simulink model "DualBuckPPS22016_define"  (R2024b)
settings: Solver=ode45  StartTime=0.0  StopTime=0.5  RelTol=1e-3
model workspace (MAT data in the model file):
  D = 50
  T = 0.0333333333333
undefined symbols (not defined in the file): C, D_T_DOWN_Given, D_T_UP_Given, DiscIntNeverNeededParam, P, R, T_pulse, TP
libraries: spsOnDelayLib x27, dspsnks4 x12, dspfdesign x11, spsCurrentMeasurementLib x11, spsSeriesRLCBranchLib x8, spsMosfetLib x4, slpidlib x4, spsVoltageMeasurementLib x4, simulink x3, spsControlledCurrentSourceLib x1, spsDCVoltageSourceLib x1, spspowerguiLib x1
(part 1 of 2)
settings Model: SimulationMode=accelerator  Creator=10474  LastModifiedBy=admin
settings SolverCC: AlgebraicLoopSolver=TrustRegion
settings OptimizationCC: ReuseModelBlockBuffer=off
settings DebuggingCC: UnconnectedInputMsg=warning  UnconnectedOutputMsg=warning  UnconnectedLineMsg=warning  ArithmeticOperatorsInVariantConditions=warning
settings ModelReferenceCC: EnableRefExpFcnMdlSchedulingChecks=on
settings SFSimCC: CustomCodeUndefinedFunction=UseInterfaceOnly
settings RTWCC: GPUComputeCapability=3.5
settings CodeAppCC: StateflowObjectComments=on

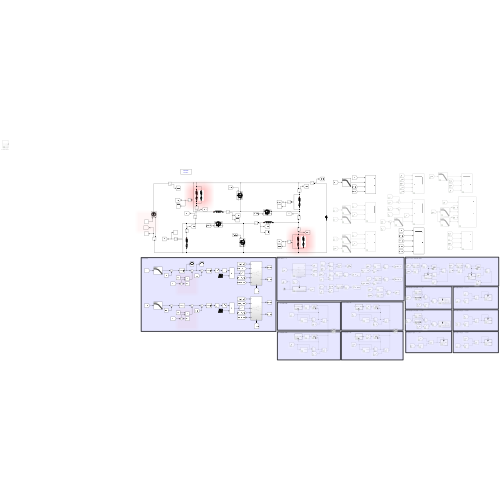
[thumbnail: Simulink's stored preview of the top-level diagram]
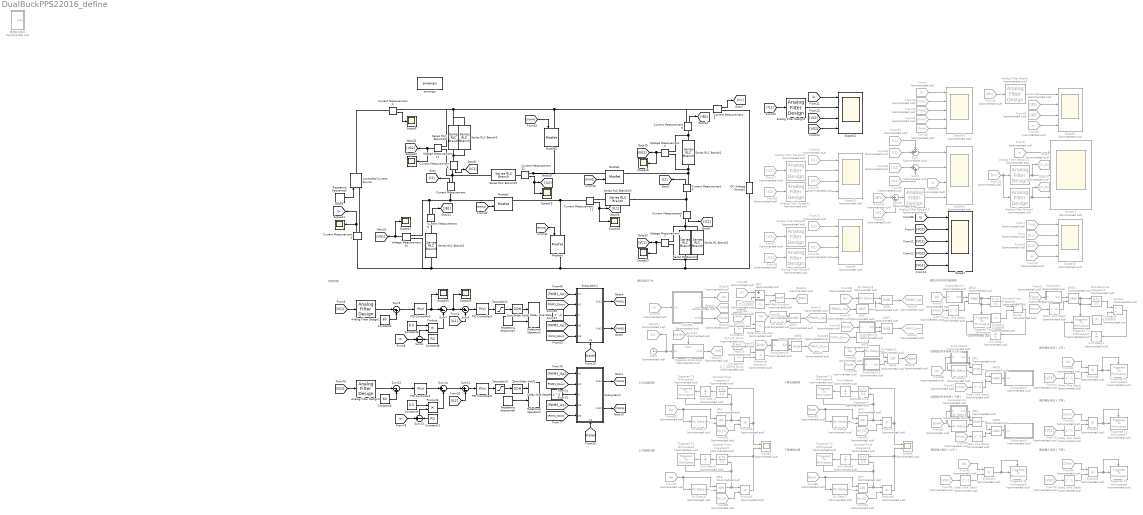
== system DualBuckPPS22016_define ==
  note: 控制回路
  note: 上升尖峰获取
  note: 上升滤除尖峰
  note: 下降尖峰获取
  note: 下降滤除尖峰
  note: 切回稳态开关采样（上升）
  note: 瞬态开关序列均值获取
  note: 切回稳态开关采样（下降）
  note: 瞬态波形产生
  note: 瞬态输入电压（下降）
  note: 瞬态输出电压（下降）
  note: 瞬态输出电压（上升）
  note: 瞬态输入电压（上升）
  AND{1..8} (8 alike) : Logic  Commented=on  IconShape=distinctive  AllPortsSameDT=off  OutDataTypeStr=boolean
  AND9 : Logic  Commented=on  Operator=OR  IconShape=distinctive  AllPortsSameDT=off  OutDataTypeStr=boolean
  Add : Sum  Commented=on  Inputs=+-
  Analog Filter Design{,5..6,10..12} (6 alike) : dspfdesign/Analog Filter Design  Commented=on  method=Butterworth  filttype=Lowpass  N=8  Wlo=2*pi*5000  Whi=80  Rp=2  Rs=40
  Analog Filter Design1 : dspfdesign/Analog Filter Design  Commented=on  method=Butterworth  filttype=Lowpass  N=2  Wlo=2*pi*1000  Whi=80  Rp=2  Rs=40
  Analog Filter Design13 : dspfdesign/Analog Filter Design  Commented=on  method=Butterworth  filttype=Lowpass  N=2  Wlo=2*pi*10000  Whi=80  Rp=2  Rs=40
  Analog Filter Design2 : dspfdesign/Analog Filter Design  method=Butterworth  filttype=Lowpass  N=1  Wlo=10  Whi=80  Rp=2  Rs=40
  Analog Filter Design3 : dspfdesign/Analog Filter Design  method=Butterworth  filttype=Lowpass  N=1  Wlo=10  Whi=80  Rp=2  Rs=40
  Analog Filter Design9 : dspfdesign/Analog Filter Design  method=Butterworth  filttype=Lowpass  N=8  Wlo=2*pi*5000  Whi=80  Rp=2  Rs=40
  Clock : Clock  Commented=on
  Constant : Constant  Commented=on  Value=1/100000
  Constant1 : Constant  Commented=on  Value=1/100000
  Constant10 : Constant  Commented=on  Value=D_T_DOWN_Given
  Constant11 : Constant  Value=P/2
  Constant2 : Constant  Commented=on  Value=D_T_UP_Given
  Constant3 : Constant  Value=60
  Constant4 : Constant  Value=60
  Constant5 : Constant  Commented=on  Value=1/100000
  Constant6 : Constant  Value=0.5
  Constant8 : Constant  Value=P/2
  Constant9 : Constant  Value=0.5
  Controlled Current Source : spsControlledCurrentSourceLib/Controlled Current Source  Initialize=on  Source_Type=DC  Amplitude=0  Phase=0  Frequency=0  Measurements=None
  Current Measurement{,1..8,11..12} (11 alike) : spsCurrentMeasurementLib/Current Measurement  PhasorSimulation=off  OutputType=Complex  PSBequivalent=0
  DC Voltage Source1 : spsDCVoltageSourceLib/DC Voltage Source  Amplitude=270  Measurements=None
  Delay One Step : Delay  DelayLength=1
  Delay One Step1 : Delay  Commented=on
  Delay One Step{2..3,5..8} (6 alike) : Delay  Commented=on  DelayLength=1
  Delay One Step4 : Delay  Commented=on
  Delay One Step9 : Delay  DelayLength=1
  Discrete-Time Integrator{,1,3..6} (6 alike) : DiscreteIntegrator  Commented=on  ExternalReset=falling  SampleTime=-1  ICPrevOutput=DiscIntNeverNeededParam  ICPrevScaledInput=DiscIntNeverNeededParam
  Divide : Product  Commented=on  Inputs=*/
  Divide1 : Product  Commented=on  Inputs=*/
  From : From  Commented=on  GotoTag=IL1
  From10 : From  Commented=on  GotoTag=IL2
  From{2,9,14,37,39,47} (6 alike) : From  Commented=on  GotoTag=io  TagVisibility=global
  From{15,25,29,41} (4 alike) : From  Commented=on  GotoTag=I1
  From16 : From  Commented=on  GotoTag=I2
  From17 : From  Commented=on  GotoTag=IC1
  From18 : From  Commented=on  GotoTag=IC2
  From19 : From  Commented=on  GotoTag=Iin
  From26 : From  Commented=on  GotoTag=I2
  From27 : From  Commented=on  GotoTag=IL1
  From28 : From  Commented=on  GotoTag=IL2
  From{3,42,55,61,66} (5 alike) : From  Commented=on  GotoTag=PWM1
  From34 : From  Commented=on  GotoTag=I2
  From35 : From  Commented=on  GotoTag=IL2
  From36 : From  Commented=on  GotoTag=IL1
  From38 : From  Commented=on  GotoTag=IB2
  From40 : From  Commented=on  GotoTag=IB1
  From43 : From  Commented=on  GotoTag=PWM2
  From44 : From  Commented=on  GotoTag=PWM3
  From45 : From  Commented=on  GotoTag=PWM4
  From46 : From  Commented=on  GotoTag=IB1
  From48 : From  Commented=on  GotoTag=IB1
  From{5,58,60,72,83,88,90,94,96} (9 alike) : From  Commented=on  GotoTag=Down  TagVisibility=global
  From54 : From  Commented=on  GotoTag=VC1
  From{56,67..69,81..82,87,92,95} (9 alike) : From  Commented=on  GotoTag=Up  TagVisibility=global
  From57 : From  Commented=on  GotoTag=PWM1_Up
  From59 : From  Commented=on  GotoTag=PWM1_Down  TagVisibility=global
  From63 : From  Commented=on  GotoTag=t0
  From64 : From  Commented=on  GotoTag=State1  TagVisibility=global
  From65 : From  Commented=on  GotoTag=t
  From7 : From  Commented=on  GotoTag=Iin
  From71 : From  Commented=on  GotoTag=MW
  From73 : From  Commented=on  GotoTag=MW
  From79 : From  Commented=on  GotoTag=VC1
  From80 : From  Commented=on  GotoTag=Iin_f1
  From84 : From  Commented=on  GotoTag=Iin_f2
  From85 : From  Commented=on  GotoTag=Iin_f1
  From89 : From  Commented=on  GotoTag=Iin_f2
  From91 : From  Commented=on  GotoTag=VG1
  From93 : From  Commented=on  GotoTag=VG1
  Goto10 : Goto  Commented=on  GotoTag=Up  TagVisibility=global
  Goto11 : Goto  Commented=on  GotoTag=State  TagVisibility=global
  Goto13 : Goto  Commented=on  GotoTag=Down  TagVisibility=global
  Goto15 : Goto  Commented=on  GotoTag=Iin_f2
  Goto16 : Goto  Commented=on  GotoTag=PWM2_Up
  Goto17 : Goto  Commented=on  GotoTag=PWM2_Down
  Goto18 : Goto  Commented=on  GotoTag=State1  TagVisibility=global
  Goto20 : Goto  Commented=on  GotoTag=t0
  Goto21 : Goto  Commented=on  GotoTag=t
  Goto22 : Goto  Commented=on  GotoTag=PWM1_Down  TagVisibility=global
  Goto23 : Goto  Commented=on  GotoTag=PWM1_Up
  Goto24 : Goto  Commented=on  GotoTag=MW
  Goto3 : Goto  Commented=on  GotoTag=Iin_f1
  Math Function : Math  Commented=on  Operator=mod
  Mosfet{1..4} (4 alike) : spsMosfetLib/Mosfet  Ron=53e-3  Lon=0  Rd=0.001  Vfd=2  IC=0  Rs=1e5  Cs=inf  Measurements=on
  NOT7 : Logic  Commented=on  Operator=NOT  IconShape=distinctive  AllPortsSameDT=off  OutDataTypeStr=boolean
  NOT8 : Logic  Commented=on  Operator=NOT  IconShape=distinctive  AllPortsSameDT=off  OutDataTypeStr=boolean
  OR2 : Logic  Commented=on  Operator=XOR  IconShape=distinctive  AllPortsSameDT=off  OutDataTypeStr=boolean
  OR3 : Logic  Commented=on  Operator=XOR  IconShape=distinctive  AllPortsSameDT=off  OutDataTypeStr=boolean
  OR{4..7} (4 alike) : Logic  Commented=on  Operator=OR  IconShape=distinctive  AllPortsSameDT=off  OutDataTypeStr=boolean
  On Delay1 : spsOnDelayLib/On Delay  Commented=on  DelayType=Off delay  delay=ceil(TP*1e5)*1e-5-TP  ic=0  Ts=0
  On Delay11 : spsOnDelayLib/On Delay  Commented=on  DelayType=Off delay  delay=ceil(TP*1e5)*1e-5-TP  ic=0  Ts=0
  On Delay12 : spsOnDelayLib/On Delay  Commented=on  DelayType=Off delay  delay=ceil(TP*1e5)*1e-5-TP  ic=0  Ts=0
  On Delay3 : spsOnDelayLib/On Delay  Commented=on  DelayType=Off delay  delay=30e-6  ic=0  Ts=0
  On Delay{4..7} (4 alike) : spsOnDelayLib/On Delay  Commented=on  DelayType=Off delay  delay=TP  ic=0  Ts=0
  On Delay9 : spsOnDelayLib/On Delay  Commented=on  DelayType=Off delay  delay=30e-6  ic=0  Ts=0
  PID Controller1 : slpidlib/PID Controller  Controller=PI  Form=Parallel  TimeDomain=Discrete-time  UseExternalTs=off  SampleTime=-1  IntegratorMethod=Forward Euler  FilterMethod=Forward Euler  ControllerParametersSource=internal  P=0.15  I=0.5  UseKiTs=off  D=0  UseExternalDerivativeSource=off  N=100  UseFilter=on  TunerSelectOption=Transfer Function Based (PID Tuner App)  InitialConditionSource=internal  InitialConditionForIntegrator=0  InitialConditionForFilter=0  DifferentiatorICPrevScaledInput=0  ExternalReset=none  TrackingMode=off  Kt=1  LimitOutput=on  SatLimitsSource=internal  UpperSaturationLimit=10  LowerSaturationLimit=-10  LinearizeAsGain=on  AntiWindupMode=none  Kb=1  LimitIntegrator=off  UpperIntegratorSaturationLimit=inf  LowerIntegratorSaturationLimit=-inf  POutMin=[]  POutMax=[]  IOutMin=[]  IOutMax=[]  DOutMin=[]  DOutMax=[]  NOutMin=[]  NOutMax=[]  SumOutMin=[]  SumOutMax=[]  SaturationOutMin=[]  SaturationOutMax=[]  PParamMin=[]  PParamMax=[]  IParamMin=[]  IParamMax=[]  DParamMin=[]  DParamMax=[]  NParamMin=[]  NParamMax=[]  KbParamMin=[]  KbParamMax=[]  KtParamMin=[]  KtParamMax=[]  KbOutMin=[]  KbOutMax=[]  KtOutMin=[]  KtOutMax=[]  IntegratorOutMin=[]  IntegratorOutMax=[]  FilterOutMin=[]  FilterOutMax=[]  SumI1OutMin=[]  SumI1OutMax=[]  SumI2OutMin=[]  SumI2OutMax=[]  SumI3OutMin=[]  SumI3OutMax=[]  SumI4OutMin=[]  SumI4OutMax=[]  SumDOutMin=[]  SumDOutMax=[]  DifferentiatorOutMin=[]  DifferentiatorOutMax=[]  FilterDiffOutCoefMin=[]  FilterDiffOutCoefMax=[]  ReciprocalOutMin=[]  ReciprocalOutMax=[]  SumDenOutMin=[]  SumDenOutMax=[]  SumNumOutMin=[]  SumNumOutMax=[]  DivideOutMin=[]  DivideOutMax=[]  UdiffTsProdOutMin=[]  UdiffTsProdOutMax=[]  NTsProdOutMin=[]  NTsProdOutMax=[]  UintegralTsProdOutMin=[]  UintegralTsProdOutMax=[]  UngainTsProdOutMin=[]  UngainTsProdOutMax=[]  ClampingZeroOutDataTypeStr=Inherit: Inherit via back propagation  ClampingZeroOutMin=[]  ClampingZeroOutMax=[]  FilterDenConstantOutDataTypeStr=Inherit: Inherit via back propagation  FilterDenConstantOutMin=[]  FilterDenConstantOutMax=[]  PCopyOutDataTypeStr=Inherit: Inherit via back propagation  PCopyOutMin=[]  PCopyOutMax=[]  NCopyOutDataTypeStr=Inherit: Inherit via back propagation  NCopyOutMin=[]  NCopyOutMax=[]  IntegratorContinuousStateAttributes=''  IntegratorStateMustResolveToSignalObject=off  IntegratorRTWStateStorageClass=Auto  FilterContinuousStateAttributes=''  FilterStateMustResolveToSignalObject=off  FilterRTWStateStorageClass=Auto  ParallelPVariant=InternalParameters  IdealPVariant=Disabled  IVariant=InternalParameters  DVariant=Disabled  IntegratorVariant=Discrete  SatVariant=Enabled  AWVariant=Passthrough  PCopyVariant=Disabled  TRVariant=Disabled  FdbkBlocksVariant=Forward  IdealPFdbkVariant=Disabled  SatFdbkVariant=Disabled  DerivativeFilterVariant=Disabled  NVariant=Disabled  NCopyVariant=Disabled_SignalSpec  FilterICVariant=Disabled  IntegratorICVariant=InternalICs  ExternalResetVariant=Disabled  TRSumVariant=Passthrough  SumFdbkVariant=Disabled  SumVariant=Sum_PI  TsampFilterVariant=InternalTs  TsampNgainVariant=Passthrough  TsampIntegralVariant=Disabled_SignalSpec  ExternalSaturationOutDataTypeStr=Inherit: Same as second input  DerivativeSourceVariant=Disabled  PreIntVariant=InternalPreInt
  PID Controller3 : slpidlib/PID Controller  Controller=PI  Form=Parallel  TimeDomain=Discrete-time  UseExternalTs=off  SampleTime=-1  IntegratorMethod=Forward Euler  FilterMethod=Forward Euler  ControllerParametersSource=internal  P=0.2  I=2  UseKiTs=off  D=0  UseExternalDerivativeSource=off  N=100  UseFilter=on  TunerSelectOption=Transfer Function Based (PID Tuner App)  InitialConditionSource=internal  InitialConditionForIntegrator=0  InitialConditionForFilter=0  DifferentiatorICPrevScaledInput=0  ExternalReset=none  TrackingMode=off  Kt=1  LimitOutput=on  SatLimitsSource=internal  UpperSaturationLimit=0.98  LowerSaturationLimit=0  LinearizeAsGain=on  AntiWindupMode=none  Kb=1  LimitIntegrator=off  UpperIntegratorSaturationLimit=inf  LowerIntegratorSaturationLimit=-inf  POutMin=[]  POutMax=[]  IOutMin=[]  IOutMax=[]  DOutMin=[]  DOutMax=[]  NOutMin=[]  NOutMax=[]  SumOutMin=[]  SumOutMax=[]  SaturationOutMin=[]  SaturationOutMax=[]  PParamMin=[]  PParamMax=[]  IParamMin=[]  IParamMax=[]  DParamMin=[]  DParamMax=[]  NParamMin=[]  NParamMax=[]  KbParamMin=[]  KbParamMax=[]  KtParamMin=[]  KtParamMax=[]  KbOutMin=[]  KbOutMax=[]  KtOutMin=[]  KtOutMax=[]  IntegratorOutMin=[]  IntegratorOutMax=[]  FilterOutMin=[]  FilterOutMax=[]  SumI1OutMin=[]  SumI1OutMax=[]  SumI2OutMin=[]  SumI2OutMax=[]  SumI3OutMin=[]  SumI3OutMax=[]  SumI4OutMin=[]  SumI4OutMax=[]  SumDOutMin=[]  SumDOutMax=[]  DifferentiatorOutMin=[]  DifferentiatorOutMax=[]  FilterDiffOutCoefMin=[]  FilterDiffOutCoefMax=[]  ReciprocalOutMin=[]  ReciprocalOutMax=[]  SumDenOutMin=[]  SumDenOutMax=[]  SumNumOutMin=[]  SumNumOutMax=[]  DivideOutMin=[]  DivideOutMax=[]  UdiffTsProdOutMin=[]  UdiffTsProdOutMax=[]  NTsProdOutMin=[]  NTsProdOutMax=[]  UintegralTsProdOutMin=[]  UintegralTsProdOutMax=[]  UngainTsProdOutMin=[]  UngainTsProdOutMax=[]  ClampingZeroOutDataTypeStr=Inherit: Inherit via back propagation  ClampingZeroOutMin=[]  ClampingZeroOutMax=[]  FilterDenConstantOutDataTypeStr=Inherit: Inherit via back propagation  FilterDenConstantOutMin=[]  FilterDenConstantOutMax=[]  PCopyOutDataTypeStr=Inherit: Inherit via back propagation  PCopyOutMin=[]  PCopyOutMax=[]  NCopyOutDataTypeStr=Inherit: Inherit via back propagation  NCopyOutMin=[]  NCopyOutMax=[]  IntegratorContinuousStateAttributes=''  IntegratorStateMustResolveToSignalObject=off  IntegratorRTWStateStorageClass=Auto  FilterContinuousStateAttributes=''  FilterStateMustResolveToSignalObject=off  FilterRTWStateStorageClass=Auto  ParallelPVariant=InternalParameters  IdealPVariant=Disabled  IVariant=InternalParameters  DVariant=Disabled  IntegratorVariant=Discrete  SatVariant=Enabled  AWVariant=Passthrough  PCopyVariant=Disabled  TRVariant=Disabled  FdbkBlocksVariant=Forward  IdealPFdbkVariant=Disabled  SatFdbkVariant=Disabled  DerivativeFilterVariant=Disabled  NVariant=Disabled  NCopyVariant=Disabled_SignalSpec  FilterICVariant=Disabled  IntegratorICVariant=InternalICs  ExternalResetVariant=Disabled  TRSumVariant=Passthrough  SumFdbkVariant=Disabled  SumVariant=Sum_PI  TsampFilterVariant=InternalTs  TsampNgainVariant=Passthrough  TsampIntegralVariant=Disabled_SignalSpec  ExternalSaturationOutDataTypeStr=Inherit: Same as second input  DerivativeSourceVariant=Disabled  PreIntVariant=InternalPreInt
  PID Controller4 : slpidlib/PID Controller  Controller=PI  Form=Parallel  TimeDomain=Discrete-time  UseExternalTs=off  SampleTime=-1  IntegratorMethod=Forward Euler  FilterMethod=Forward Euler  ControllerParametersSource=internal  P=0.15  I=0.5  UseKiTs=off  D=0  UseExternalDerivativeSource=off  N=100  UseFilter=on  TunerSelectOption=Transfer Function Based (PID Tuner App)  InitialConditionSource=internal  InitialConditionForIntegrator=0  InitialConditionForFilter=0  DifferentiatorICPrevScaledInput=0  ExternalReset=none  TrackingMode=off  Kt=1  LimitOutput=off  SatLimitsSource=internal  UpperSaturationLimit=1  LowerSaturationLimit=-1  LinearizeAsGain=on  AntiWindupMode=none  Kb=1  LimitIntegrator=off  UpperIntegratorSaturationLimit=inf  LowerIntegratorSaturationLimit=-inf  POutMin=[]  POutMax=[]  IOutMin=[]  IOutMax=[]  DOutMin=[]  DOutMax=[]  NOutMin=[]  NOutMax=[]  SumOutMin=[]  SumOutMax=[]  SaturationOutMin=[]  SaturationOutMax=[]  PParamMin=[]  PParamMax=[]  IParamMin=[]  IParamMax=[]  DParamMin=[]  DParamMax=[]  NParamMin=[]  NParamMax=[]  KbParamMin=[]  KbParamMax=[]  KtParamMin=[]  KtParamMax=[]  KbOutMin=[]  KbOutMax=[]  KtOutMin=[]  KtOutMax=[]  IntegratorOutMin=[]  IntegratorOutMax=[]  FilterOutMin=[]  FilterOutMax=[]  SumI1OutMin=[]  SumI1OutMax=[]  SumI2OutMin=[]  SumI2OutMax=[]  SumI3OutMin=[]  SumI3OutMax=[]  SumI4OutMin=[]  SumI4OutMax=[]  SumDOutMin=[]  SumDOutMax=[]  DifferentiatorOutMin=[]  DifferentiatorOutMax=[]  FilterDiffOutCoefMin=[]  FilterDiffOutCoefMax=[]  ReciprocalOutMin=[]  ReciprocalOutMax=[]  SumDenOutMin=[]  SumDenOutMax=[]  SumNumOutMin=[]  SumNumOutMax=[]  DivideOutMin=[]  DivideOutMax=[]  UdiffTsProdOutMin=[]  UdiffTsProdOutMax=[]  NTsProdOutMin=[]  NTsProdOutMax=[]  UintegralTsProdOutMin=[]  UintegralTsProdOutMax=[]  UngainTsProdOutMin=[]  UngainTsProdOutMax=[]  ClampingZeroOutDataTypeStr=Inherit: Inherit via back propagation  ClampingZeroOutMin=[]  ClampingZeroOutMax=[]  FilterDenConstantOutDataTypeStr=Inherit: Inherit via back propagation  FilterDenConstantOutMin=[]  FilterDenConstantOutMax=[]  PCopyOutDataTypeStr=Inherit: Inherit via back propagation  PCopyOutMin=[]  PCopyOutMax=[]  NCopyOutDataTypeStr=Inherit: Inherit via back propagation  NCopyOutMin=[]  NCopyOutMax=[]  IntegratorContinuousStateAttributes=''  IntegratorStateMustResolveToSignalObject=off  IntegratorRTWStateStorageClass=Auto  FilterContinuousStateAttributes=''  FilterStateMustResolveToSignalObject=off  FilterRTWStateStorageClass=Auto  ParallelPVariant=InternalParameters  IdealPVariant=Disabled  IVariant=InternalParameters  DVariant=Disabled  IntegratorVariant=Discrete  SatVariant=Disabled  AWVariant=Passthrough  PCopyVariant=Disabled  TRVariant=Disabled  FdbkBlocksVariant=Forward  IdealPFdbkVariant=Disabled  SatFdbkVariant=Disabled  DerivativeFilterVariant=Disabled  NVariant=Disabled  NCopyVariant=Disabled_SignalSpec  FilterICVariant=Disabled  IntegratorICVariant=InternalICs  ExternalResetVariant=Disabled  TRSumVariant=Passthrough  SumFdbkVariant=Disabled  SumVariant=Sum_PI  TsampFilterVariant=InternalTs  TsampNgainVariant=Passthrough  TsampIntegralVariant=Disabled_SignalSpec  ExternalSaturationOutDataTypeStr=Inherit: Same as second input  DerivativeSourceVariant=Disabled  PreIntVariant=InternalPreInt
  PID Controller5 : slpidlib/PID Controller  Controller=PI  Form=Parallel  TimeDomain=Discrete-time  UseExternalTs=off  SampleTime=-1  IntegratorMethod=Forward Euler  FilterMethod=Forward Euler  ControllerParametersSource=internal  P=0.2  I=2  UseKiTs=off  D=0  UseExternalDerivativeSource=off  N=100  UseFilter=on  TunerSelectOption=Transfer Function Based (PID Tuner App)  InitialConditionSource=internal  InitialConditionForIntegrator=0  InitialConditionForFilter=0  DifferentiatorICPrevScaledInput=0  ExternalReset=none  TrackingMode=off  Kt=1  LimitOutput=on  SatLimitsSource=internal  UpperSaturationLimit=0.98  LowerSaturationLimit=0  LinearizeAsGain=on  AntiWindupMode=none  Kb=1  LimitIntegrator=off  UpperIntegratorSaturationLimit=inf  LowerIntegratorSaturationLimit=-inf  POutMin=[]  POutMax=[]  IOutMin=[]  IOutMax=[]  DOutMin=[]  DOutMax=[]  NOutMin=[]  NOutMax=[]  SumOutMin=[]  SumOutMax=[]  SaturationOutMin=[]  SaturationOutMax=[]  PParamMin=[]  PParamMax=[]  IParamMin=[]  IParamMax=[]  DParamMin=[]  DParamMax=[]  NParamMin=[]  NParamMax=[]  KbParamMin=[]  KbParamMax=[]  KtParamMin=[]  KtParamMax=[]  KbOutMin=[]  KbOutMax=[]  KtOutMin=[]  KtOutMax=[]  IntegratorOutMin=[]  IntegratorOutMax=[]  FilterOutMin=[]  FilterOutMax=[]  SumI1OutMin=[]  SumI1OutMax=[]  SumI2OutMin=[]  SumI2OutMax=[]  SumI3OutMin=[]  SumI3OutMax=[]  SumI4OutMin=[]  SumI4OutMax=[]  SumDOutMin=[]  SumDOutMax=[]  DifferentiatorOutMin=[]  DifferentiatorOutMax=[]  FilterDiffOutCoefMin=[]  FilterDiffOutCoefMax=[]  ReciprocalOutMin=[]  ReciprocalOutMax=[]  SumDenOutMin=[]  SumDenOutMax=[]  SumNumOutMin=[]  SumNumOutMax=[]  DivideOutMin=[]  DivideOutMax=[]  UdiffTsProdOutMin=[]  UdiffTsProdOutMax=[]  NTsProdOutMin=[]  NTsProdOutMax=[]  UintegralTsProdOutMin=[]  UintegralTsProdOutMax=[]  UngainTsProdOutMin=[]  UngainTsProdOutMax=[]  ClampingZeroOutDataTypeStr=Inherit: Inherit via back propagation  ClampingZeroOutMin=[]  ClampingZeroOutMax=[]  FilterDenConstantOutDataTypeStr=Inherit: Inherit via back propagation  FilterDenConstantOutMin=[]  FilterDenConstantOutMax=[]  PCopyOutDataTypeStr=Inherit: Inherit via back propagation  PCopyOutMin=[]  PCopyOutMax=[]  NCopyOutDataTypeStr=Inherit: Inherit via back propagation  NCopyOutMin=[]  NCopyOutMax=[]  IntegratorContinuousStateAttributes=''  IntegratorStateMustResolveToSignalObject=off  IntegratorRTWStateStorageClass=Auto  FilterContinuousStateAttributes=''  FilterStateMustResolveToSignalObject=off  FilterRTWStateStorageClass=Auto  ParallelPVariant=InternalParameters  IdealPVariant=Disabled  IVariant=InternalParameters  DVariant=Disabled  IntegratorVariant=Discrete  SatVariant=Enabled  AWVariant=Passthrough  PCopyVariant=Disabled  TRVariant=Disabled  FdbkBlocksVariant=Forward  IdealPFdbkVariant=Disabled  SatFdbkVariant=Disabled  DerivativeFilterVariant=Disabled  NVariant=Disabled  NCopyVariant=Disabled_SignalSpec  FilterICVariant=Disabled  IntegratorICVariant=InternalICs  ExternalResetVariant=Disabled  TRSumVariant=Passthrough  SumFdbkVariant=Disabled  SumVariant=Sum_PI  TsampFilterVariant=InternalTs  TsampNgainVariant=Passthrough  TsampIntegralVariant=Disabled_SignalSpec  ExternalSaturationOutDataTypeStr=Inherit: Same as second input  DerivativeSourceVariant=Disabled  PreIntVariant=InternalPreInt
  Product : Product
  Product{1..2,4..9} (8 alike) : Product  Commented=on
  Product3 : Product
  Relational Operator : RelationalOperator  Commented=on  Operator=<  OutDataTypeStr=boolean  RndMeth=Simplest  InputSameDT=off
  Relational Operator2 : RelationalOperator  OutDataTypeStr=boolean  RndMeth=Simplest  InputSameDT=off
  Relational Operator3 : RelationalOperator  OutDataTypeStr=boolean  RndMeth=Simplest  InputSameDT=off
  Relational Operator5 : RelationalOperator  Commented=on  Operator=<  OutDataTypeStr=boolean  RndMeth=Simplest  InputSameDT=off
  Repeating Sequence1 : simulink/Sources/Repeating Sequence  rep_seq_t=[0 1/100000]  rep_seq_y=[0 1]
  Repeating Sequence3 : simulink/Sources/Repeating Sequence  rep_seq_t=[0 TP T_pulse/2+TP T_pulse/2+2*TP T_pulse]  rep_seq_y=[0 P P 0 0]
  Repeating Sequence5 : simulink/Sources/Repeating Sequence  rep_seq_t=[0 1/100000]  rep_seq_y=[0 1]
  Saturation1 : Saturate  UpperLimit=0.98  LowerLimit=0
  Saturation3 : Saturate  UpperLimit=0.98  LowerLimit=0
  Scope{6,8,10,13..14} (5 alike) : Scope  Commented=on  NumInputPorts=4
  Scope{9,11,16,18..19,21..23,29..30} (10 alike) : Scope
  Scope12 : Scope  NumInputPorts=4
  Scope15 : Scope  Commented=on  NumInputPorts=5
  Scope17 : Scope  Commented=on  NumInputPorts=3
  Scope2 : Scope  Commented=on  NumInputPorts=2
  Scope3 : Scope  Commented=on  NumInputPorts=2
  Scope7 : Scope  NumInputPorts=5
  Series RL Branch1 : spsSeriesRLCBranchLib/Series RLC Branch  LConnTagsString=__new0  RConnTagsString=__new0  BranchType=RC  Resistance=R  Inductance=1e-3  SetiL0=off  InitialCurrent=0  Capacitance=C  Setx0=on  InitialVoltage=12  Measurements=None
  Series RL Branch2 : spsSeriesRLCBranchLib/Series RLC Branch  LConnTagsString=__new0  RConnTagsString=__new0  BranchType=RC  Resistance=R  Inductance=1e-3  SetiL0=off  InitialCurrent=0  Capacitance=C  Setx0=on  InitialVoltage=12  Measurements=None
  Series RLC Branch1 : spsSeriesRLCBranchLib/Series RLC Branch  LConnTagsString=__new0  RConnTagsString=__new0  BranchType=RC  Resistance=0.001  Inductance=1e-3  SetiL0=off  InitialCurrent=0  Capacitance=2.48e-3  Setx0=on  InitialVoltage=12  Measurements=None
  Series RLC Branch18 : spsSeriesRLCBranchLib/Series RLC Branch  LConnTagsString=__new0  RConnTagsString=__new0  BranchType=RC  Resistance=R  Inductance=1e-3  SetiL0=off  InitialCurrent=0  Capacitance=C  Setx0=on  InitialVoltage=12  Measurements=None
  Series RLC Branch19 : spsSeriesRLCBranchLib/Series RLC Branch  LConnTagsString=__new0  RConnTagsString=__new0  BranchType=L  Resistance=0.01  Inductance=260e-6  SetiL0=off  InitialCurrent=15  Capacitance=1e-3  Setx0=off  InitialVoltage=0  Measurements=None
  Series RLC Branch2 : spsSeriesRLCBranchLib/Series RLC Branch  LConnTagsString=__new0  RConnTagsString=__new0  BranchType=RC  Resistance=0.2  Inductance=1e-3  SetiL0=off  InitialCurrent=0  Capacitance=2.48e-3  Setx0=on  InitialVoltage=12  Measurements=None
  Series RLC Branch20 : spsSeriesRLCBranchLib/Series RLC Branch  LConnTagsString=__new0  RConnTagsString=__new0  BranchType=L  Resistance=0.01  Inductance=260e-6  SetiL0=off  InitialCurrent=5  Capacitance=1e-3  Setx0=off  InitialVoltage=0  Measurements=None
  Series RLC Branch3 : spsSeriesRLCBranchLib/Series RLC Branch  LConnTagsString=__new0  RConnTagsString=__new0  BranchType=RC  Resistance=R  Inductance=1e-3  SetiL0=off  InitialCurrent=0  Capacitance=C  Setx0=on  InitialVoltage=12  Measurements=None
  Subsystem : Subsystem  Commented=on
  Subsystem1 : Subsystem
      settings: PortSchema="{\"entries\":[{\"content\":{\"sides\":[{\"content\":{\"connectorIds\":[\"In1\",\"In2\",\"In3\",\"In4\",\"In5\"]},\"type\":\"ConnectorPlacement.EquallySpacedRectSide\",\"uuid\":\"12f56cea-dd87-479d-8ac5-f677a0a856ab\"},{\"content\":{\"connectorIds\":[\"Out1\",\"Out2\"],\"side\":\"RIGHT\"},\"type\":\"ConnectorPlacement.EquallySpacedRectSide\",\"uuid\":\"93daadb0-c8ef-4d9e-87ae-a550f970c223\"},{\"content\":{\"side\":\"TOP\"},\"type\":\"ConnectorPlacement.EquallySpacedRectSide\",\"uuid\":\"18f26d28-3d48-45f0-84e1-51e7663a8b99\"},{\"content\":{\"connectorIds\":[\"In6\"],\"side\":\"BOTTOM\"},\"type\":\"ConnectorPlacement.EquallySpacedRectSide\",\"uuid\":\"53ae5f66-9a34-49e2-9ad8-502cdcf805c1\"}]},\"type\":\"ConnectorPlacement.EquallySpacedConnector\",\"uuid\":\"751889f7-46a5-4d64-ba57-d2d7ffe777e8\"}],\"packageUris\":[\"http://schema.mathworks.com/mf0/Connector/R2020b\"],\"version\":\"1.0\"}"
  Subsystem10 : Subsystem  Commented=on
  Subsystem11 : Subsystem  Commented=on
  Subsystem12 : Subsystem  Commented=on
  Subsystem13 : Subsystem  Commented=on
  Subsystem15 : Subsystem  Commented=on
  Subsystem2 : Subsystem
      settings: PortSchema="{\"entries\":[{\"content\":{\"sides\":[{\"content\":{\"connectorIds\":[\"In1\",\"In2\",\"In3\",\"In4\",\"In5\"]},\"type\":\"ConnectorPlacement.EquallySpacedRectSide\",\"uuid\":\"12f56cea-dd87-479d-8ac5-f677a0a856ab\"},{\"content\":{\"connectorIds\":[\"Out1\",\"Out2\"],\"side\":\"RIGHT\"},\"type\":\"ConnectorPlacement.EquallySpacedRectSide\",\"uuid\":\"93daadb0-c8ef-4d9e-87ae-a550f970c223\"},{\"content\":{\"side\":\"TOP\"},\"type\":\"ConnectorPlacement.EquallySpacedRectSide\",\"uuid\":\"18f26d28-3d48-45f0-84e1-51e7663a8b99\"},{\"content\":{\"connectorIds\":[\"In6\"],\"side\":\"BOTTOM\"},\"type\":\"ConnectorPlacement.EquallySpacedRectSide\",\"uuid\":\"53ae5f66-9a34-49e2-9ad8-502cdcf805c1\"}]},\"type\":\"ConnectorPlacement.EquallySpacedConnector\",\"uuid\":\"751889f7-46a5-4d64-ba57-d2d7ffe777e8\"}],\"packageUris\":[\"http://schema.mathworks.com/mf0/Connector/R2020b\"],\"version\":\"1.0\"}"
  Subsystem4 : Subsystem  Commented=on
  Subsystem5 : Subsystem  Commented=on
  Subsystem9 : Subsystem  Commented=on
  Sum : Sum  Commented=on  Inputs=++|
  Sum{1,7,11,14} (4 alike) : Sum  Inputs=|+-
  Sum10 : Sum  Commented=on  Inputs=|+-
  Sum12 : Sum  Inputs=|-+
  Sum13 : Sum  Inputs=+-
  Sum5 : Sum  Inputs=|-+
  Sum6 : Sum  Inputs=+-
  Sum9 : Sum  Commented=on  Inputs=|++
  Triggered Subsystem : Subsystem  Commented=on  TreatAsAtomicUnit=on
  Triggered To Workspace : dspsnks4/Triggered To Workspace  Commented=on  TriggerType=Falling edge  VariableName=PWM_T_UP  Buffer=1000  Save2DMode=2-D array (concatenate along first dimension)
      settings: FixptAsFi=off
  Triggered To Workspace1 : dspsnks4/Triggered To Workspace  Commented=on  TriggerType=Falling edge  VariableName=PWM_T_DOWN  Buffer=1000  Save2DMode=2-D array (concatenate along first dimension)
      settings: FixptAsFi=off
  Triggered To Workspace2 : dspsnks4/Triggered To Workspace  Commented=on  TriggerType=Falling edge  VariableName=Iin_Pulse_UP  Buffer=1000  Save2DMode=2-D array (concatenate along first dimension)
      settings: FixptAsFi=off
  Triggered To Workspace3 : dspsnks4/Triggered To Workspace  Commented=on  TriggerType=Rising edge  VariableName=VC1_UP  Buffer=1000  Save2DMode=2-D array (concatenate along first dimension)
      settings: FixptAsFi=off
  Triggered To Workspace4 : dspsnks4/Triggered To Workspace  Commented=on  TriggerType=Falling edge  VariableName=Iin_Pulse_DOWN  Buffer=1000  Save2DMode=2-D array (concatenate along first dimension)
      settings: FixptAsFi=off
  Triggered To Workspace5 : dspsnks4/Triggered To Workspace  Commented=on  TriggerType=Falling edge  VariableName=Iin_Pulse_UP_ref  Buffer=1000  Save2DMode=2-D array (concatenate along first dimension)
      settings: FixptAsFi=off
  Triggered To Workspace6 : dspsnks4/Triggered To Workspace  Commented=on  TriggerType=Falling edge  VariableName=Iin_Pulse_DOWN_ref  Buffer=1000  Save2DMode=2-D array (concatenate along first dimension)
      settings: FixptAsFi=off
  Triggered To Workspace7 : dspsnks4/Triggered To Workspace  Commented=on  TriggerType=Rising edge  VariableName=VC1_DOWN  Buffer=1000  Save2DMode=2-D array (concatenate along first dimension)
      settings: FixptAsFi=off
  Triggered To Workspace8 : dspsnks4/Triggered To Workspace  Commented=on  TriggerType=Rising edge  VariableName=VG1_DOWN  Buffer=1000  Save2DMode=2-D array (concatenate along first dimension)
      settings: FixptAsFi=off
  Triggered To Workspace9 : dspsnks4/Triggered To Workspace  Commented=on  TriggerType=Rising edge  VariableName=VG1_UP  Buffer=1000  Save2DMode=2-D array (concatenate along first dimension)
      settings: FixptAsFi=off
  Unit Delay{,1,3..6} (6 alike) : UnitDelay  Commented=on  SampleTime=-1  HasFrameUpgradeWarning=on
  Voltage Measurement{2,7,10..11} (4 alike) : spsVoltageMeasurementLib/Voltage Measurement  PhasorSimulation=off  OutputType=Complex  PSBequivalent=0
  Zero-Order Hold : ZeroOrderHold  SampleTime=1e-5
  Zero-Order Hold1 : ZeroOrderHold  SampleTime=1e-5
  powergui : spspowerguiLib/powergui  Priority=1  SimulationMode=Discrete  SampleTime=1e-7  frequency=60  Iterations=50  frequencyindice=0  Pbase=100e6  ErrMax=1e-4  UnitsV=kV  UnitsW=MW  buscounter=0  FunctionMessages=off  echomessages=off  EnableUseOfTLC=off  CurrentSourceSwitches=off  DisableSnubberDevices=off  DisableRonSwitches=off  DisableVfSwitches=off  DisplayEquations=off  AutomaticDiscreteSolvers=off  SolverType=Tustin/Backward Euler (TBE)  Interpol=off  ExternalGateDelay=off  methode=off  Ts=100  x0status=blocks  SPID=on  SwTol=0  HookPort=off  NonlinearTolerance=1e-4  nMaxIteration=100  ContinueOnMaxIteration=off  RestoreLinks=warning  ResistiveCurrentMeasurement=off  Frange=[0:2:500]  Ylog=off  Xlog=on  ShowGrid=off  save=off  variable=ZData  structure=0  ZoomFFT=off  StartTime=0.0  cycles=1  DisplayStyle=1  fundamental=60  FreqAxis=off  MaxFrequency=1000  frequencyindicesteady=1  RmsSteady=1  display=off
  状态判断 : Subsystem  Commented=on
  理想脉冲输出 : Subsystem  Commented=on
  tag scope: io=global
  wires:
  [PWM2] -> Mosfet4/1
  Current Measurement12/1 -> Scope19/1, [IL2]
  [PWM4] -> Mosfet3/1
  Current Measurement11/1 -> Scope18/1, [IL1]
  Voltage Measurement10/1 -> Scope21/1, [VG1]
  [PWM1] -> Mosfet2/1
  Voltage Measurement11/1 -> Scope22/1, [VC2]
  Current Measurement8/1 -> [IB2]
  Current Measurement2/1 -> Scope11/1, [io]
  [VC1] -> Analog Filter Design2/1
  Analog Filter Design2/1 -> Sum5/1
  Sum5/1 -> PID Controller1/1
  Repeating Sequence1/1 -> Relational Operator2/2
  Constant4/1 -> Sum5/2
  [PWM3] -> Mosfet1/1
  Current Measurement1/1 -> Scope9/1
  Current Measurement3/1 -> [Iin]
  PID Controller3/1 -> Saturation1/1
  Sum1/1 -> PID Controller3/1
  PID Controller1/1 -> Scope29/1, Sum7/1
  [io] -> Sum6/1
  Sum7/1 -> Scope30/1, Sum1/1
  Sum6/1 -> Product/2
  Product/1 -> Sum7/2
  Constant6/1 -> Product/1
  [IL1] -> Sum1/2
  Constant8/1 -> Sum6/2
  Current Measurement/1 -> [I1]
  Current Measurement4/1 -> [I2]
  Current Measurement6/1 -> [IC1]
  Current Measurement7/1 -> [IC2]
  Repeating Sequence3/1 -> Controlled Current Source/1
  Current Measurement5/1 -> [IB1]
  Voltage Measurement7/1 -> Scope23/1, [VC1]
  Voltage Measurement2/1 -> [VG2], Scope16/1
  Subsystem1/2(Out2) -> [PWM2]
  [PWM2_Down] -> Subsystem1/5(In6)
  [PWM2_Up] -> Subsystem1/4(In5)
  [State1] -> Subsystem1/6(In3)
  [PWM1_Down] -> Subsystem1/2(In2)
  [PWM1_Up] -> Subsystem1/1(In1)
  Subsystem1/1(Out1) -> [PWM1]
  Saturation3/1 -> Zero-Order Hold1/1
  Subsystem2/1(Out1) -> [PWM3]
  [PWM1_Up] -> Subsystem2/1(In1)
  [PWM1_Down] -> Subsystem2/2(In2)
  [State1] -> Subsystem2/6(In3)
  [PWM2_Up] -> Subsystem2/4(In5)
  [PWM2_Down] -> Subsystem2/5(In6)
  Subsystem2/2(Out2) -> [PWM4]
  Constant11/1 -> Sum13/2
  [IL2] -> Sum11/2
  Constant9/1 -> Product3/1
  Product3/1 -> Sum14/2
  Sum13/1 -> Product3/2
  Sum14/1 -> Sum11/1
  [io] -> Sum13/1
  PID Controller4/1 -> Sum14/1
  Sum11/1 -> PID Controller5/1
  PID Controller5/1 -> Saturation3/1
  Constant3/1 -> Sum12/2
  Repeating Sequence5/1 -> Relational Operator3/2
  Sum12/1 -> PID Controller4/1
  Analog Filter Design3/1 -> Sum12/1
  [VC2] -> Analog Filter Design3/1
  Saturation1/1 -> Zero-Order Hold/1
  Zero-Order Hold/1 -> Relational Operator2/1
  Zero-Order Hold1/1 -> Relational Operator3/1
  [io] -> Scope12/1
  [io] -> Scope7/1
  Analog Filter Design12/1 -> Scope13/4
  From36/1 -> Sum9/2
  From15/1 -> Scope8/1
  From28/1 -> Analog Filter Design12/1
  From45/1 -> Scope15/5
  [VG1] -> Scope7/5
  From48/1 -> Scope6/2
  From14/1 -> Scope10/4
  Analog Filter Design/1 -> Scope6/1
  From29/1 -> Sum/1
  From38/1 -> Scope6/3
  [VC1] -> Scope7/3
  From/1 -> Scope10/2
  From27/1 -> Analog Filter Design11/1
  From37/1 -> Scope14/3
  From43/1 -> Scope15/3
  From39/1 -> Scope6/4
  From19/1 -> Analog Filter Design1/1, Analog Filter Design13/1
  Analog Filter Design1/1 -> Scope17/3, Goto15/1
  From2/1 -> Scope15/1
  Sum/1 -> Scope14/1
  [VC2] -> Scope12/3
  Analog Filter Design5/1 -> Scope8/2
  From44/1 -> Scope15/4
  [VG2] -> Scope12/4
  [VG2] -> Scope7/4
  From26/1 -> Scope13/3
  [IL1] -> Analog Filter Design9/1
  From41/1 -> Sum10/2
  [VC2] -> Scope7/2
  Sum10/1 -> Analog Filter Design10/1
  From40/1 -> Sum10/1
  Analog Filter Design9/1 -> Scope12/2
  From10/1 -> Scope10/3
  From34/1 -> Sum/2
  From18/1 -> Analog Filter Design6/1
  Analog Filter Design13/1 -> Scope17/2, Goto3/1
  From46/1 -> Analog Filter Design/1
  Analog Filter Design6/1 -> Scope8/4
  From9/1 -> Scope17/1
  From42/1 -> Scope15/2
  Sum9/1 -> Scope14/2
  Analog Filter Design11/1 -> Scope13/2
  Analog Filter Design10/1 -> Scope14/4
  From7/1 -> Scope10/1
  From35/1 -> Sum9/1
  From16/1 -> Scope8/3
  From25/1 -> Scope13/1
  From17/1 -> Analog Filter Design5/1
  On Delay7/1 -> OR7/2
  Unit Delay3/1 -> Triggered To Workspace2/1
  Discrete-Time Integrator4/1 -> Unit Delay4/1
  On Delay5/1 -> OR5/2
  Product7/1 -> Discrete-Time Integrator4/1, Scope3/1
  OR4/1 -> Product2/1, Triggered To Workspace2/Trigger, Discrete-Time Integrator3/2
  Discrete-Time Integrator6/1 -> Unit Delay6/1
  From84/1 -> Product8/2
  Unit Delay5/1 -> Triggered To Workspace5/1
  OR7/1 -> Product8/1, Discrete-Time Integrator6/2, Triggered To Workspace6/Trigger
  Product8/1 -> Scope3/2, Discrete-Time Integrator6/1
  Unit Delay4/1 -> Triggered To Workspace4/1
  From80/1 -> Product7/2
  Discrete-Time Integrator5/1 -> Unit Delay5/1
  OR6/1 -> Discrete-Time Integrator5/2, Triggered To Workspace5/Trigger, Product5/1
  From83/1 -> OR5/1, On Delay5/1
  Product5/1 -> Scope2/2, Discrete-Time Integrator5/1
  Unit Delay6/1 -> Triggered To Workspace6/1
  From85/1 -> Product2/2
  OR5/1 -> Triggered To Workspace4/Trigger, Discrete-Time Integrator4/2, Product7/1
  From87/1 -> OR6/1, On Delay6/1
  On Delay6/1 -> OR6/2
  From88/1 -> On Delay7/1, OR7/1
  On Delay4/1 -> OR4/2
  Product2/1 -> Discrete-Time Integrator3/1, Scope2/1
  Discrete-Time Integrator3/1 -> Unit Delay3/1
  From89/1 -> Product5/2
  From82/1 -> On Delay4/1, OR4/1
  Delay One Step1/1 -> AND5/2
  Subsystem11/1(Out) -> OR2/1, On Delay9/1
  Delay One Step4/1 -> AND8/2
  From68/1 -> Subsystem9/1(In)
  Delay One Step3/1 -> AND2/2
  Divide/1 -> Unit Delay/1
  From3/1 -> Delay One Step2/1
  Discrete-Time Integrator/1 -> Divide/1
  From55/1 -> Delay One Step4/1
  Subsystem9/1(Out) -> OR3/1, On Delay3/1
  Subsystem/1(Out) -> AND4/1
  OR3/1 -> AND5/1
  From61/1 -> Delay One Step1/1
  AND2/1 -> Triggered To Workspace/Trigger, Discrete-Time Integrator/2, Discrete-Time Integrator/1
  On Delay3/1 -> OR3/2
  AND8/1 -> Subsystem5/1(In1)
  Divide1/1 -> Unit Delay1/1
  From66/1 -> Delay One Step3/1
  From60/1 -> Subsystem11/1(In)
  Delay One Step2/1 -> AND4/2
  Constant5/1 -> Divide1/2
  Unit Delay1/1 -> Triggered To Workspace1/1
  AND4/1 -> Discrete-Time Integrator1/2, Triggered To Workspace1/Trigger, Discrete-Time Integrator1/1
  Discrete-Time Integrator1/1 -> Divide1/1
  OR2/1 -> AND8/1
  Unit Delay/1 -> Triggered To Workspace/1
  On Delay9/1 -> OR2/2
  From5/1 -> Subsystem/1(In)
  AND5/1 -> Subsystem4/1(In1)
  From67/1 -> Subsystem10/1(In)
  Subsystem10/1(Out) -> AND2/1
  Constant/1 -> Divide/2
  Relational Operator/1 -> AND1/2
  From95/1 -> On Delay11/1
  AND3/1 -> Goto22/1
  From69/1 -> On Delay1/1
  From96/1 -> Subsystem13/1(In)
  On Delay11/1 -> AND9/1
  From56/1 -> On Delay12/1
  Subsystem12/1(Out) -> AND3/1
  On Delay12/1 -> AND6/1
  AND9/1 -> Goto18/1
  Subsystem15/1(Out) -> AND7/1
  Math Function/1 -> Goto24/1
  Relational Operator5/1 -> AND3/2
  AND1/1 -> Goto23/1
  From57/1 -> NOT7/1
  状态判断/2(Out2) -> Goto11/1
  From72/1 -> Subsystem12/1(In)
  Clock/1 -> Triggered Subsystem/1(In1), Goto21/1
  NOT7/1 -> AND6/2
  From64/1 -> Triggered Subsystem/Trigger
  Triggered Subsystem/1(Out1) -> Goto20/1
  Constant10/1 -> Relational Operator5/2
  Constant1/1 -> Math Function/2
  From71/1 -> Relational Operator/1
  AND6/1 -> Goto16/1
  From58/1 -> Subsystem15/1(In)
  状态判断/1(y) -> Goto10/1
  From73/1 -> Relational Operator5/1
  NOT8/1 -> AND7/2
  状态判断/3(Out3) -> Goto13/1
  From59/1 -> NOT8/1
  On Delay1/1 -> AND1/1
  From65/1 -> Add/1
  From63/1 -> Add/2
  AND7/1 -> Goto17/1
  Subsystem13/1(Out) -> AND9/2
  From47/1 -> 状态判断/1(In1)
  Add/1 -> Math Function/1
  Constant2/1 -> Relational Operator/2
  Relational Operator2/1 -> Delay One Step/1
  Delay One Step/1 -> Subsystem1/3(In)
  Relational Operator3/1 -> Delay One Step9/1
  Delay One Step9/1 -> Subsystem2/3(In)
  Product6/1 -> Triggered To Workspace3/1, Triggered To Workspace3/Trigger
  Product1/1 -> Triggered To Workspace7/Trigger, Triggered To Workspace7/1
  From90/1 -> Product1/1
  From93/1 -> Delay One Step8/1
  Delay One Step8/1 -> Product9/2
  From94/1 -> Product9/1
  Delay One Step6/1 -> Product1/2
  Delay One Step5/1 -> Product6/2
  From79/1 -> Delay One Step6/1
  Product9/1 -> Triggered To Workspace8/1, Triggered To Workspace8/Trigger
  From81/1 -> Product6/1
  From54/1 -> Delay One Step5/1
  From91/1 -> Delay One Step7/1
  From92/1 -> Product4/1
  Delay One Step7/1 -> Product4/2
  Product4/1 -> Triggered To Workspace9/Trigger, Triggered To Workspace9/1
  connections:
  Series RL Branch1/RConn1 -- Series RL Branch2/RConn1 -- Voltage Measurement7/LConn2 -- DC Voltage Source1/LConn1 -- Mosfet4/RConn1 -- Voltage Measurement10/LConn2 -- Current Measurement2/LConn1 -- Series RLC Branch2/RConn1
  Current Measurement8/RConn1 -- Current Measurement3/LConn1 -- Mosfet3/LConn1 -- Series RLC Branch3/LConn1 -- Series RLC Branch18/LConn1 -- Current Measurement1/RConn1 -- Voltage Measurement11/LConn1
  Current Measurement12/RConn1 -- Mosfet3/RConn1 -- Mosfet1/LConn1
  Current Measurement11/RConn1 -- Series RLC Branch20/LConn1
  Series RLC Branch20/RConn1 -- Current Measurement7/LConn1 -- Current Measurement4/LConn1
  Current Measurement12/LConn1 -- Series RLC Branch19/RConn1
  Series RLC Branch19/LConn1 -- Voltage Measurement11/LConn2 -- Current Measurement/RConn1 -- Current Measurement6/RConn1
  Series RLC Branch1/LConn1 -- Current Measurement8/LConn1 -- Voltage Measurement2/LConn1
  Current Measurement2/RConn1 -- Controlled Current Source/LConn1
  Current Measurement1/LConn1 -- Controlled Current Source/RConn1
  Current Measurement3/RConn1 -- DC Voltage Source1/RConn1
  Current Measurement5/LConn1 -- Series RLC Branch2/LConn1
  Current Measurement4/RConn1 -- Mosfet1/RConn1 -- Voltage Measurement2/LConn2 -- Series RLC Branch1/RConn1
  Current Measurement7/RConn1 -- Series RL Branch2/LConn1 -- Voltage Measurement7/LConn1 -- Series RL Branch1/LConn1
  Series RLC Branch18/RConn1 -- Series RLC Branch3/RConn1 -- Current Measurement6/LConn1
  Mosfet4/LConn1 -- Mosfet2/RConn1 -- Current Measurement11/LConn1
  Current Measurement/LConn1 -- Current Measurement5/RConn1 -- Voltage Measurement10/LConn1 -- Mosfet2/LConn1

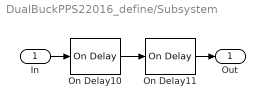
== system DualBuckPPS22016_define/Subsystem ==
  In : Inport
  On Delay10 : spsOnDelayLib/On Delay  DelayType=On delay  delay=ceil(TP*1e5)*1e-5-TP  ic=0  Ts=0
  On Delay11 : spsOnDelayLib/On Delay  DelayType=Off delay  delay=ceil((TP-(ceil(TP*1e5)*1e-5-TP))*1e5)*1e-5-(TP-(ceil(TP*1e5)*1e-5-TP))  ic=0  Ts=0
  Out : Outport
  wires:
  On Delay10/1 -> On Delay11/1
  In/1 -> On Delay10/1
  On Delay11/1 -> Out/1

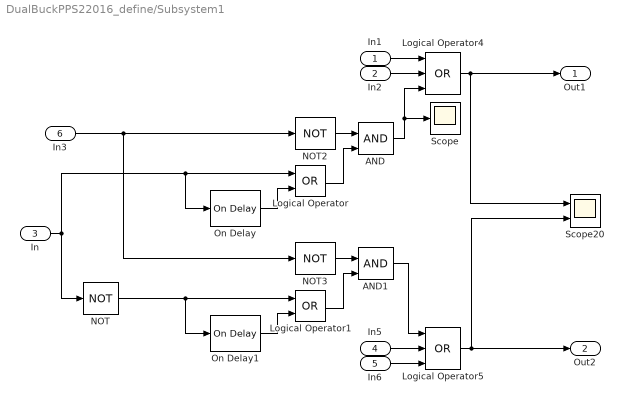
== system DualBuckPPS22016_define/Subsystem1 ==
  In1 : Inport
  In2 : Inport  Port=2
  In : Inport  Port=3
  In5 : Inport  Port=4
  In6 : Inport  Port=5
  In3 : Inport  Port=6
  AND : Logic  IconShape=distinctive  AllPortsSameDT=off  OutDataTypeStr=boolean
  AND1 : Logic  IconShape=distinctive  AllPortsSameDT=off  OutDataTypeStr=boolean
  Logical Operator : Logic  Operator=OR  AllPortsSameDT=off  OutDataTypeStr=boolean
  Logical Operator1 : Logic  Operator=OR  AllPortsSameDT=off  OutDataTypeStr=boolean
  Logical Operator4 : Logic  Operator=OR  Inputs=3  AllPortsSameDT=off  OutDataTypeStr=boolean
  Logical Operator5 : Logic  Operator=OR  Inputs=3  AllPortsSameDT=off  OutDataTypeStr=boolean
  NOT : Logic  Operator=NOT  IconShape=distinctive  AllPortsSameDT=off  OutDataTypeStr=boolean
  NOT2 : Logic  Operator=NOT  IconShape=distinctive  AllPortsSameDT=off  OutDataTypeStr=boolean
  NOT3 : Logic  Operator=NOT  IconShape=distinctive  AllPortsSameDT=off  OutDataTypeStr=boolean
  On Delay : spsOnDelayLib/On Delay  DelayType=On delay  delay=100e-9  ic=0  Ts=0
  On Delay1 : spsOnDelayLib/On Delay  DelayType=On delay  delay=100e-9  ic=0  Ts=0
  Scope : Scope
  Scope20 : Scope  NumInputPorts=2
  Out1 : Outport
  Out2 : Outport  Port=2
  wires:
  In5/1 -> Logical Operator5/2
  In6/1 -> Logical Operator5/3
  In3/1 -> NOT3/1, NOT2/1
  In/1 -> Logical Operator/1, On Delay/1, NOT/1
  NOT2/1 -> AND/1
  NOT3/1 -> AND1/1
  Logical Operator1/1 -> AND1/2
  NOT/1 -> Logical Operator1/1, On Delay1/1
  Logical Operator5/1 -> Scope20/2, Out2/1
  Logical Operator4/1 -> Scope20/1, Out1/1
  In2/1 -> Logical Operator4/2
  On Delay/1 -> Logical Operator/2
  On Delay1/1 -> Logical Operator1/2
  AND1/1 -> Logical Operator5/1
  AND/1 -> Logical Operator4/3, Scope/1
  Logical Operator/1 -> AND/2
  In1/1 -> Logical Operator4/1

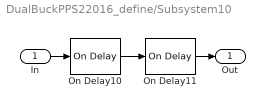
== system DualBuckPPS22016_define/Subsystem10 ==
  In : Inport
  On Delay10 : spsOnDelayLib/On Delay  DelayType=On delay  delay=10e-6  ic=0  Ts=0
  On Delay11 : spsOnDelayLib/On Delay  DelayType=Off delay  delay=ceil(TP*1e5)*1e-5-TP  ic=0  Ts=0
  Out : Outport
  wires:
  On Delay11/1 -> Out/1
  In/1 -> On Delay10/1
  On Delay10/1 -> On Delay11/1

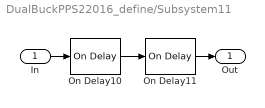
== system DualBuckPPS22016_define/Subsystem11 ==
  In : Inport
  On Delay10 : spsOnDelayLib/On Delay  DelayType=On delay  delay=ceil(TP*1e5)*1e-5-TP  ic=0  Ts=0
  On Delay11 : spsOnDelayLib/On Delay  DelayType=Off delay  delay=ceil((TP-(ceil(TP*1e5)*1e-5-TP))*1e5)*1e-5-(TP-(ceil(TP*1e5)*1e-5-TP))  ic=0  Ts=0
  Out : Outport
  wires:
  On Delay10/1 -> On Delay11/1
  In/1 -> On Delay10/1
  On Delay11/1 -> Out/1

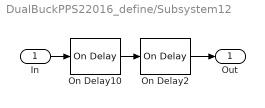
== system DualBuckPPS22016_define/Subsystem12 ==
  In : Inport
  On Delay10 : spsOnDelayLib/On Delay  DelayType=On delay  delay=ceil(TP*1e5)*1e-5-TP  ic=0  Ts=0
  On Delay2 : spsOnDelayLib/On Delay  DelayType=Off delay  delay=ceil((TP-(ceil(TP*1e5)*1e-5-TP))*1e5)*1e-5-(TP-(ceil(TP*1e5)*1e-5-TP))  ic=0  Ts=0
  Out : Outport
  wires:
  On Delay2/1 -> Out/1
  In/1 -> On Delay10/1
  On Delay10/1 -> On Delay2/1

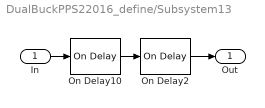
== system DualBuckPPS22016_define/Subsystem13 ==
  In : Inport
  On Delay10 : spsOnDelayLib/On Delay  DelayType=On delay  delay=ceil(TP*1e5)*1e-5-TP  ic=0  Ts=0
  On Delay2 : spsOnDelayLib/On Delay  DelayType=Off delay  delay=ceil((TP-(ceil(TP*1e5)*1e-5-TP))*1e5)*1e-5-(TP-(ceil(TP*1e5)*1e-5-TP))  ic=0  Ts=0
  Out : Outport
  wires:
  On Delay10/1 -> On Delay2/1
  In/1 -> On Delay10/1
  On Delay2/1 -> Out/1

== system DualBuckPPS22016_define/Subsystem15 ==
  In : Inport
  On Delay10 : spsOnDelayLib/On Delay  DelayType=On delay  delay=ceil(TP*1e5)*1e-5-TP  ic=0  Ts=0
  On Delay2 : spsOnDelayLib/On Delay  DelayType=Off delay  delay=ceil((TP-(ceil(TP*1e5)*1e-5-TP))*1e5)*1e-5-(TP-(ceil(TP*1e5)*1e-5-TP))  ic=0  Ts=0
  Out : Outport
  wires:
  On Delay10/1 -> On Delay2/1
  In/1 -> On Delay10/1
  On Delay2/1 -> Out/1

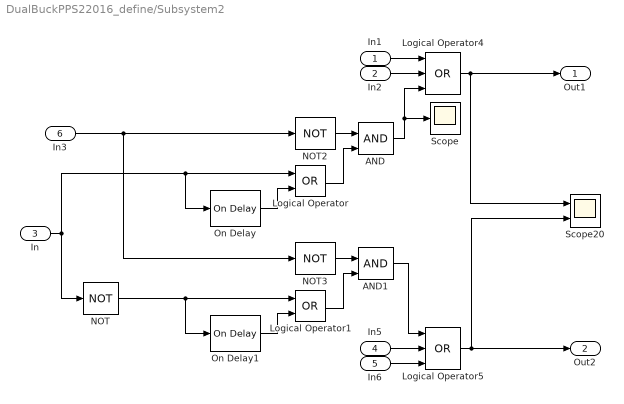
== system DualBuckPPS22016_define/Subsystem2 ==
  In1 : Inport
  In2 : Inport  Port=2
  In : Inport  Port=3
  In5 : Inport  Port=4
  In6 : Inport  Port=5
  In3 : Inport  Port=6
  AND : Logic  IconShape=distinctive  AllPortsSameDT=off  OutDataTypeStr=boolean
  AND1 : Logic  IconShape=distinctive  AllPortsSameDT=off  OutDataTypeStr=boolean
  Logical Operator : Logic  Operator=OR  AllPortsSameDT=off  OutDataTypeStr=boolean
  Logical Operator1 : Logic  Operator=OR  AllPortsSameDT=off  OutDataTypeStr=boolean
  Logical Operator4 : Logic  Operator=OR  Inputs=3  AllPortsSameDT=off  OutDataTypeStr=boolean
  Logical Operator5 : Logic  Operator=OR  Inputs=3  AllPortsSameDT=off  OutDataTypeStr=boolean
  NOT : Logic  Operator=NOT  IconShape=distinctive  AllPortsSameDT=off  OutDataTypeStr=boolean
  NOT2 : Logic  Operator=NOT  IconShape=distinctive  AllPortsSameDT=off  OutDataTypeStr=boolean
  NOT3 : Logic  Operator=NOT  IconShape=distinctive  AllPortsSameDT=off  OutDataTypeStr=boolean
  On Delay : spsOnDelayLib/On Delay  DelayType=On delay  delay=100e-9  ic=0  Ts=0
  On Delay1 : spsOnDelayLib/On Delay  DelayType=On delay  delay=100e-9  ic=0  Ts=0
  Scope : Scope
  Scope20 : Scope  NumInputPorts=2
  Out1 : Outport
  Out2 : Outport  Port=2
  wires:
  In1/1 -> Logical Operator4/1
  Logical Operator/1 -> AND/2
  AND/1 -> Scope/1, Logical Operator4/3
  AND1/1 -> Logical Operator5/1
  On Delay1/1 -> Logical Operator1/2
  On Delay/1 -> Logical Operator/2
  In2/1 -> Logical Operator4/2
  Logical Operator4/1 -> Out1/1, Scope20/1
  Logical Operator5/1 -> Out2/1, Scope20/2
  NOT/1 -> On Delay1/1, Logical Operator1/1
  Logical Operator1/1 -> AND1/2
  NOT3/1 -> AND1/1
  NOT2/1 -> AND/1
  In/1 -> NOT/1, On Delay/1, Logical Operator/1
  In3/1 -> NOT2/1, NOT3/1
  In6/1 -> Logical Operator5/3
  In5/1 -> Logical Operator5/2

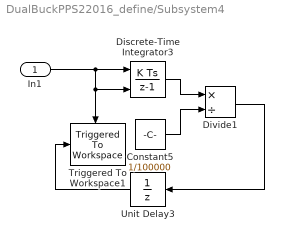
== system DualBuckPPS22016_define/Subsystem4 ==
  In1 : Inport
  Constant5 : Constant  Value=1/100000
  Discrete-Time Integrator3 : DiscreteIntegrator  ExternalReset=falling  SampleTime=-1  ICPrevOutput=DiscIntNeverNeededParam  ICPrevScaledInput=DiscIntNeverNeededParam
  Divide1 : Product  Inputs=*/
  Triggered To Workspace1 : dspsnks4/Triggered To Workspace  TriggerType=Falling edge  VariableName=PWM_S_UP  Buffer=1000  Save2DMode=2-D array (concatenate along first dimension)
      settings: FixptAsFi=off
  Unit Delay3 : UnitDelay  SampleTime=-1  HasFrameUpgradeWarning=on
  wires:
  Divide1/1 -> Unit Delay3/1
  Constant5/1 -> Divide1/2
  In1/1 -> Triggered To Workspace1/Trigger, Discrete-Time Integrator3/2, Discrete-Time Integrator3/1
  Discrete-Time Integrator3/1 -> Divide1/1
  Unit Delay3/1 -> Triggered To Workspace1/1

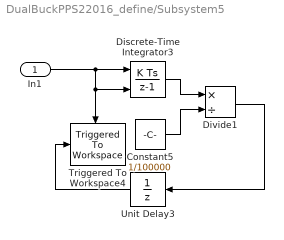
== system DualBuckPPS22016_define/Subsystem5 ==
  In1 : Inport
  Constant5 : Constant  Value=1/100000
  Discrete-Time Integrator3 : DiscreteIntegrator  ExternalReset=falling  SampleTime=-1  ICPrevOutput=DiscIntNeverNeededParam  ICPrevScaledInput=DiscIntNeverNeededParam
  Divide1 : Product  Inputs=*/
  Triggered To Workspace4 : dspsnks4/Triggered To Workspace  TriggerType=Falling edge  VariableName=PWM_S_DOWN  Buffer=1000  Save2DMode=2-D array (concatenate along first dimension)
      settings: FixptAsFi=off
  Unit Delay3 : UnitDelay  SampleTime=-1  HasFrameUpgradeWarning=on
  wires:
  Unit Delay3/1 -> Triggered To Workspace4/1
  Discrete-Time Integrator3/1 -> Divide1/1
  Constant5/1 -> Divide1/2
  Divide1/1 -> Unit Delay3/1
  In1/1 -> Discrete-Time Integrator3/1, Triggered To Workspace4/Trigger, Discrete-Time Integrator3/2

== system DualBuckPPS22016_define/Subsystem9 ==
  In : Inport
  On Delay10 : spsOnDelayLib/On Delay  DelayType=On delay  delay=10e-6  ic=0  Ts=0
  On Delay11 : spsOnDelayLib/On Delay  DelayType=Off delay  delay=ceil(TP*1e5)*1e-5-TP  ic=0  Ts=0
  Out : Outport
  wires:
  On Delay10/1 -> On Delay11/1
  In/1 -> On Delay10/1
  On Delay11/1 -> Out/1

== system DualBuckPPS22016_define/Triggered Subsystem ==
  In1 : Inport
  Trigger : TriggerPort  VariantControl=(inherit)
  Out1 : Outport
  wires:
  In1/1 -> Out1/1

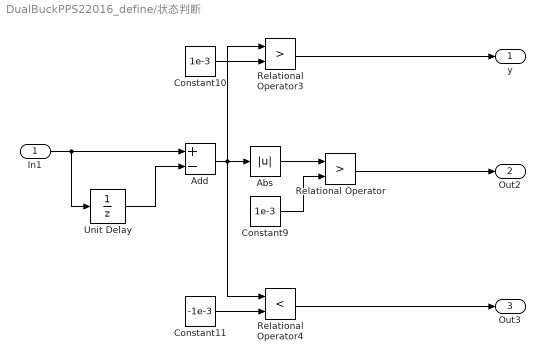
== system DualBuckPPS22016_define/状态判断 ==
  In1 : Inport
  Abs : Abs  SaturateOnIntegerOverflow=off
  Add : Sum  Inputs=+-
  Constant10 : Constant  Value=1e-3
  Constant11 : Constant  Value=-1e-3
  Constant9 : Constant  Value=1e-3
  Relational Operator : RelationalOperator  Operator=>  OutDataTypeStr=boolean  RndMeth=Simplest  InputSameDT=off
  Relational Operator3 : RelationalOperator  Operator=>  OutDataTypeStr=boolean  RndMeth=Simplest  InputSameDT=off
  Relational Operator4 : RelationalOperator  Operator=<  OutDataTypeStr=boolean  RndMeth=Simplest  InputSameDT=off
  Unit Delay : UnitDelay  SampleTime=-1  HasFrameUpgradeWarning=on
  y : Outport
  Out2 : Outport  Port=2
  Out3 : Outport  Port=3
  wires:
  In1/1 -> Unit Delay/1, Add/1
  Constant10/1 -> Relational Operator3/2
  Unit Delay/1 -> Add/2
  Constant9/1 -> Relational Operator/2
  Constant11/1 -> Relational Operator4/2
  Add/1 -> Relational Operator4/1, Relational Operator3/1, Abs/1
  Abs/1 -> Relational Operator/1
  Relational Operator3/1 -> y/1
  Relational Operator/1 -> Out2/1
  Relational Operator4/1 -> Out3/1
